simulink model "mod_ofdm"  (R2024b)
settings: Solver=FixedStepDiscrete  StartTime=0.0  StopTime=1  FixedStep=8.0000000000000007e-05  RelTol=1e-3
model workspace (MAT data in the model file):
  ND = 48
  NS = 80
  Tsym = 8e-05
  graines_I = [387516902 1591540660 907041352 915802074 1362320394 1122932516 890960854 3064203 198131879 1523412860 1126023594 1494993211 2051852598 1466546334 114092995 663256090 1272587400 504917230 2072259441 2029475606 1821927017 1014308058 1807057484 281557961 663000481 994277185 1593104732 1043301734 293939227 737739080 696699894 645144684 355411551 890994772 962331784 1664085885 1710236006 1121824257 989196028 1671200983 1905438514 1449377021 1719015667 2016726274 87307686 1880490709 593914676 1021696482 1711031125 1540265965 315997005 1414651113 148717688 766803335 1745538166 918489135 1288177595 1563714448 1763572859 1633193783 15340067 902494678 994577455 119184276 1162738124 1305177750 1779089688 2022520002 275195421 494846105 1415531878 284485725 481205209 1234508006 364049424 1679826458 1840341143 72314804 1143846008 1711440007]
  graines_Q = [2094096518 588965844 363141769 1882700910 1952454473 424198650 948177902 1544539262 1815364904 361368467 1428009973 1734813438 1180502085 353726331 76297528 604589270 1734889431 96134814 17644811 776565838 136627819 321019392 49800937 1126827269 1496143057 917090393 288987860 711584192 1267758068 2020054959 2131501470 518838313 22720178 1783786516 1989886131 984843473 1656659819 1860148260 1309137810 1873952605 51331358 583246294 595324521 259056167 1955742250 65367828 1444313812 153200812 774770211 897861931 389562745 1118869267 1148886058 680846552 1582884554 344032057 413408252 761306614 812556559 442995504 1972912994 1778317398 229516061 793464962 499657373 968683923 593386639 1077622093 1981275183 821436416 1396139954 1279086600 1614807976 132425289 1599496659 2032112079 1296134267 617573223 1443901901 1529113125]
  graines_src = [163870804 1674862852 941476655 1553629638 2100216483 1156411076 1076148001 154728631 576468320 1073489496 1458635309 1726016436 818064854 141597227 618787963 1953337226 458241558 970928814 1999749699 53470684 1289668979 2040387564 494571667 1177873132 1952338318 285979207 1124019958 1611492901 1436694994 1004491617 439910072 1053911721 799690031 1025211173 785743620 1799415190 1650657950 674298435 1229703538 592810817 972472792 758015269 1411754596 795322894 985894663 1544736790 886893199 1946529147]
  ptsI = [0.707106781187 -0.707106781187 -0.707106781187 0.707106781187]
  ptsQ = [0.707106781187 0.707106781187 -0.707106781187 -0.707106781187]
  sigma2 = 0
  taps = 1
settings Model: Creator=runner  LastModifiedBy=runner

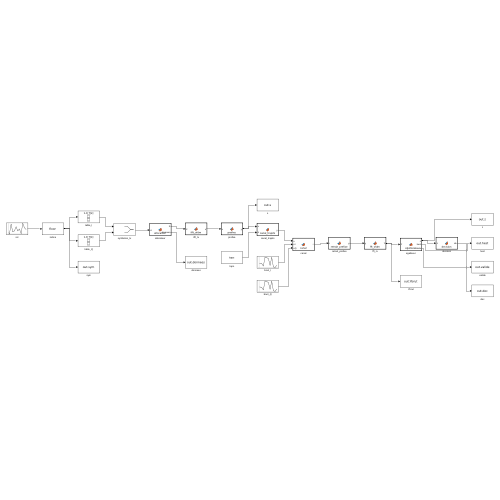
[thumbnail: Simulink's stored preview of the top-level diagram]
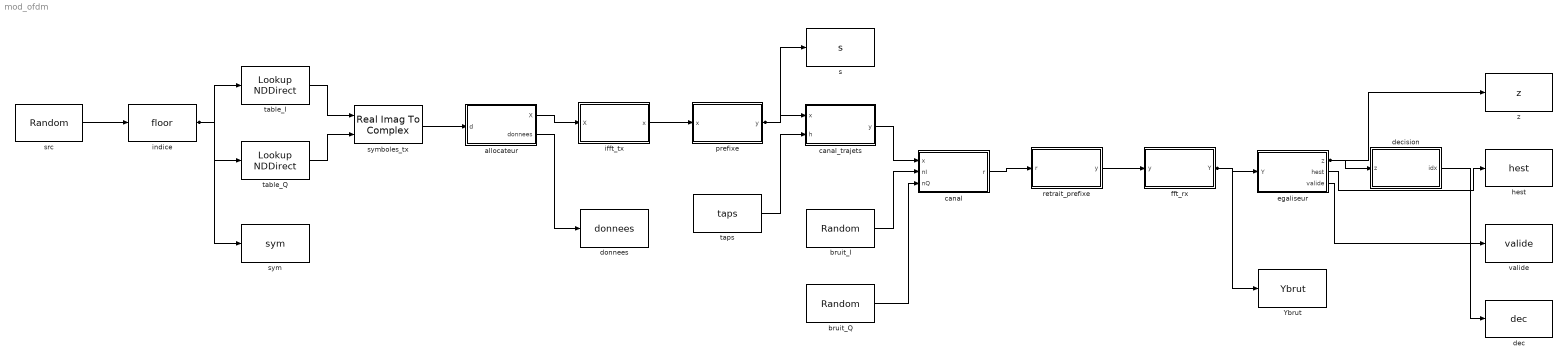
== system mod_ofdm ==
  Ybrut : ToWorkspace  VariableName=Ybrut  SampleTime=-1
  allocateur : MATLAB Function  TreatAsAtomicUnit=on
  bruit_I : RandomNumber  Mean=zeros(1, NS)  Variance=sigma2 / 2  Seed=graines_I  SampleTime=Tsym
  bruit_Q : RandomNumber  Mean=zeros(1, NS)  Variance=sigma2 / 2  Seed=graines_Q  SampleTime=Tsym
  canal : MATLAB Function  TreatAsAtomicUnit=on
  canal_trajets : MATLAB Function  TreatAsAtomicUnit=on
  dec : ToWorkspace  VariableName=dec  SampleTime=-1
  decision : MATLAB Function  TreatAsAtomicUnit=on
  donnees : ToWorkspace  VariableName=donnees  SampleTime=-1
  egaliseur : MATLAB Function  TreatAsAtomicUnit=on
  fft_rx : MATLAB Function  TreatAsAtomicUnit=on
  hest : ToWorkspace  VariableName=hest  SampleTime=-1
  ifft_tx : MATLAB Function  TreatAsAtomicUnit=on
  indice : Rounding
  prefixe : MATLAB Function  TreatAsAtomicUnit=on
  retrait_prefixe : MATLAB Function  TreatAsAtomicUnit=on
  s : ToWorkspace  VariableName=s  SampleTime=-1
  src : UniformRandomNumber  Minimum=zeros(1, ND)  Maximum=4 * ones(1, ND)  Seed=graines_src  SampleTime=Tsym
  sym : ToWorkspace  VariableName=sym  SampleTime=-1
  symboles_tx : RealImagToComplex
  table_I : LookupNDDirect  NumberOfTableDimensions=1  Table=ptsI
  table_Q : LookupNDDirect  NumberOfTableDimensions=1  Table=ptsQ
  taps : Constant  Value=taps
  valide : ToWorkspace  VariableName=valide  SampleTime=-1
  z : ToWorkspace  VariableName=z  SampleTime=-1
  wires:
  src/1 -> indice/1
  indice/1 -> table_I/1, table_Q/1, sym/1
  table_I/1 -> symboles_tx/1
  table_Q/1 -> symboles_tx/2
  symboles_tx/1 -> allocateur/1(d)
  allocateur/1(X) -> ifft_tx/1(X)
  allocateur/2(donnees) -> donnees/1
  ifft_tx/1(x) -> prefixe/1(x)
  prefixe/1(y) -> s/1, canal_trajets/1(x)
  taps/1 -> canal_trajets/2(h)
  canal_trajets/1(y) -> canal/1(x)
  bruit_I/1 -> canal/2(nI)
  bruit_Q/1 -> canal/3(nQ)
  canal/1(r) -> retrait_prefixe/1(r)
  retrait_prefixe/1(y) -> fft_rx/1(y)
  fft_rx/1(Y) -> egaliseur/1(Y), Ybrut/1
  egaliseur/1(z) -> decision/1(z), z/1
  egaliseur/2(hest) -> hest/1
  egaliseur/3(valide) -> valide/1
  decision/1(idx) -> dec/1

== matlab function mod_ofdm/allocateur ==
  data: d input; X output; donnees output
function [X, donnees] = allocateur(d)
% repartition sur les porteuses (porteuse 0 a l'indice 33) : 2 symboles d'apprentissage puis 20 symboles
% de donnees par trame, 48 porteuses de donnees et 4 pilotes (equivalent du bloc OFDM Carrier Allocator)
persistent k
if isempty(k), k = 0; end
pre = [0 0 0 0 0 0 -1 1 1 -1 -1 -1 -1 -1 1 1 1 -1 1 -1 1 -1 1 -1 1 1 -1 1 1 -1 -1 -1 0 -1 -1 -1 -1 1 1 -1 -1 -1 1 1 1 -1 1 1 -1 1 -1 1 1 1 1 -1 -1 -1 1 0 0 0 0 0];
occ = [7 8 9 10 11 13 14 15 16 17 18 19 20 21 22 23 24 25 27 28 29 30 31 32 34 35 36 37 38 39 41 42 43 44 45 46 47 48 49 50 51 52 53 55 56 57 58 59];
pil = [12 26 40 54];
pils = [1 1 1 -1];
X = complex(zeros(1, 64));
if k < 2
    X = complex(pre); donnees = 0;
else
    d = d(:).'; X(occ) = d; X(pil) = pils; donnees = 1;
end
k = k + 1; if k == 22, k = 0; end
end

== matlab function mod_ofdm/prefixe ==
  data: x input; y output
function y = prefixe(x)
% prefixe cyclique : copie des 16 derniers echantillons en tete du symbole
x = x(:).'; y = [x(49:64), x];
end

== matlab function mod_ofdm/canal_trajets ==
  data: x input; y output; h input
function y = canal_trajets(x, h)
% canal a trajets multiples : filtre a reponse impulsionnelle finie de coefficients h, avec memoire
% d'un symbole OFDM au suivant (equivalent du bloc FIR Filter)
persistent mem
h = h(:).'; x = x(:).'; L = numel(h);
if isempty(mem), mem = complex(zeros(1, max(L - 1, 1))); end
u = [mem(1:L - 1), x]; y = complex(zeros(1, numel(x)));
for n = 1:numel(x)
    acc = complex(0);
    for k = 1:L
        acc = acc + h(k) * u(n + L - k);
    end
    y(n) = acc;
end
if L > 1, mem(1:L - 1) = u(end - L + 2:end); end
end

== matlab function mod_ofdm/canal ==
  data: x input; r output; nI input; nQ input
function r = canal(x, nI, nQ)
% addition du bruit gaussien complexe
r = x(:).' + complex(nI(:).', nQ(:).');
end

== matlab function mod_ofdm/retrait_prefixe ==
  data: r input; y output
function y = retrait_prefixe(r)
% retrait du prefixe cyclique (equivalent du bloc Keep M in N)
r = r(:).'; y = r(17:80);
end

== matlab function mod_ofdm/fft_rx ==
  data: y input; Y output
function Y = fft_ofdm(y)
% FFT non normalisee, porteuse 0 au centre en sortie
Y = fftshift(fft(y(:).'));
end

== matlab function mod_ofdm/egaliseur ==
  data: Y input; z output; hest output; valide output
function [z, hest, valide] = egaliseur(Y)
% estimation du canal par la moyenne des 2 symboles d'apprentissage, puis egalisation Z = Y / H
% sur chaque porteuse et extraction des 48 porteuses de donnees (meme code que le bloc Python de GNU Radio)
persistent k acc h
if isempty(k), k = 0; acc = complex(zeros(1, 64)); h = complex(ones(1, 64)); end
pre = [0 0 0 0 0 0 -1 1 1 -1 -1 -1 -1 -1 1 1 1 -1 1 -1 1 -1 1 -1 1 1 -1 1 1 -1 -1 -1 0 -1 -1 -1 -1 1 1 -1 -1 -1 1 1 1 -1 1 1 -1 1 -1 1 1 1 1 -1 -1 -1 1 0 0 0 0 0];
used = [7 8 9 10 11 12 13 14 15 16 17 18 19 20 21 22 23 24 25 26 27 28 29 30 31 32 34 35 36 37 38 39 40 41 42 43 44 45 46 47 48 49 50 51 52 53 54 55 56 57 58 59];
occ = [7 8 9 10 11 13 14 15 16 17 18 19 20 21 22 23 24 25 27 28 29 30 31 32 34 35 36 37 38 39 41 42 43 44 45 46 47 48 49 50 51 52 53 55 56 57 58 59];
Y = Y(:).'; z = complex(zeros(1, 48)); valide = 0;
if k < 2
    acc = acc + Y;
    if k == 1
        h = complex(ones(1, 64)); h(used) = acc(used) / 2 ./ pre(used);
    end
else
    zz = Y ./ h; z = zz(occ); valide = 1;
end
hest = h;
k = k + 1; if k == 22, k = 0; acc = complex(zeros(1, 64)); end
end

== matlab function mod_ofdm/decision ==
  data: z input; idx output
function idx = decision(z)
% decision au plus proche point de la constellation QPSK (Constellation Decoder)
pts = complex([0.70710678118654746 -0.70710678118654746 -0.70710678118654746 0.70710678118654746], [0.70710678118654746 0.70710678118654746 -0.70710678118654746 -0.70710678118654746]);
z = z(:).'; idx = zeros(1, numel(z));
for i = 1:numel(z)
    [~, m] = min(abs(z(i) - pts)); idx(i) = m - 1;
end
end

== matlab function mod_ofdm/ifft_tx ==
  data: X input; x output
function x = ifft_ofdm(X)
% IFFT non normalisee, porteuse 0 au centre en entree (comme le bloc FFT inverse de GNU Radio)
x = 64 * ifft(ifftshift(X(:).'));
end
